simulink model "simulated_model"  (R2016a)
settings: Solver=FixedStepAuto  StartTime=0.0  StopTime=7  FixedStep=0.01  RelTol=1e-3
values from neighbouring files (symbols this model uses):
  A = rolmipvar(A_vertices, 'A', N, 1)    [LMI_TCC.m]    (also in TCC_simulated_model.m = A_list{i})
  B = [D_m ... (first row only)    [LMI_TCC.m]    (also in TCC_simulated_model.m)
  C = [c_m, c_b, c_o]    [LMI_TCC.m]    (also in TCC_simulated_model.m)
  Ki = rolmipvar(nu, ny, 'Ki', 'full', N, 0)    [LMI_TCC.m]    (also in TCC_simulated_model.m = 2.2578)
  Kp = rolmipvar(nu, ny, 'Kp', 'full', N, 0)    [LMI_TCC.m]    (also in TCC_simulated_model.m = -16.6825)
  r_val = 15    [TCC_simulated_model.m]
settings Model: Creator=Melvin  LastModifiedBy=Melvin

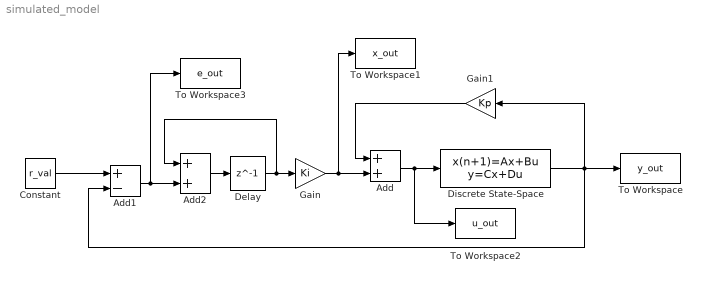
== system simulated_model ==
  Add : Sum
  Add1 : Sum  Inputs=+-
  Add2 : Sum
  Constant : Constant  Value=r_val  SampleTime=0.01
  Delay : Delay  DelayLength=1
  Discrete State-Space : DiscreteStateSpace  A=A  B=B  C=C  D=0  X0=[0 0 0]'  SampleTime=0.01
  Gain : Gain  Gain=Ki
  Gain1 : Gain  Gain=Kp
  To Workspace : ToWorkspace  VariableName=y_out  SaveFormat=Timeseries  SampleTime=-1
  To Workspace1 : ToWorkspace  VariableName=x_out  SaveFormat=Timeseries  SampleTime=-1
  To Workspace2 : ToWorkspace  VariableName=u_out  SaveFormat=Timeseries  SampleTime=-1
  To Workspace3 : ToWorkspace  VariableName=e_out  SaveFormat=Timeseries  SampleTime=-1
  wires:
  Delay/1 -> Add2/1, Gain/1
  Gain/1 -> To Workspace1/1, Add/2
  Add/1 -> To Workspace2/1, Discrete State-Space/1
  Gain1/1 -> Add/1
  Discrete State-Space/1 -> To Workspace/1, Add1/2, Gain1/1
  Constant/1 -> Add1/1
  Add2/1 -> Delay/1
  Add1/1 -> To Workspace3/1, Add2/2
